simulink model "demoDPThrusterModels"  (R2022a)
settings: Solver=ode45  StartTime=0.0  StopTime=200  RelTol=1e-3  EnableMultiTasking=on
undefined symbols (not defined in the file): slcm
libraries: mssSimulink x2, simulink_extras x2
settings Model: Creator=thor  LastModifiedBy=thor
settings SolverCC: AlgebraicLoopSolver=TrustRegion
settings DataIOCC: LimitDataPoints=on  SaveFormat=Array  SignalLoggingSaveFormat=ModelDataLogs  ReturnWorkspaceOutputs=off  SignalLoggingName=sigsOut
settings OptimizationCC: InitFltsAndDblsToZero=on  LifeSpan=inf
settings DebuggingCC: SaveWithParameterizedLinksMsg=none  UnderspecifiedInitializationDetection=Classic  MergeDetectMultiDrivingBlocksExec=none  SignalResolutionControl=TryResolveAllWithWarning  MultiTaskDSMMsg=warning  MultiTaskCondExecSysMsg=none  FcnCallInpInsideContextMsg=warning  UnconnectedInputMsg=warning  UnconnectedOutputMsg=warning  UnconnectedLineMsg=warning  SFUnexpectedBacktrackingDiag=warning  SFNoUnconditionalDefaultTransitionDiag=warning  SFExecutionAtInitializationDiag=none  SFMachineParentedDataDiag=warning  ArithmeticOperatorsInVariantConditions=warning
settings HardwareCC: ProdBitPerPointer=32  ProdBitPerSizeT=32  ProdBitPerPtrDiffT=32  ProdLargestAtomicFloat=None  ProdIntDivRoundTo=Undefined  ProdEndianess=Unspecified  ProdWordSize=32  ProdHWDeviceType=32-bit Generic  TargetUnknown=on
settings ModelReferenceCC: PropagateSignalLabelsOutOfModel=off
settings RTWCC: DLArmComputeVersion=19.05
settings CodeAppCC: StateflowObjectComments=on
settings GRTTargetCC: TargetFcnLib=ansi_tfl_tmw.mat  TargetLangStandard=C89/C90 (ANSI)  ModelReferenceCompliant=off  CombineOutputUpdateFcns=off  MatFileLogging=off  GRTInterface=on
settings ConfigComp: CovMetricSettings=dw  CovSaveCumulativeToWorkspaceVar=on  CovSaveSingleToWorkspaceVar=on

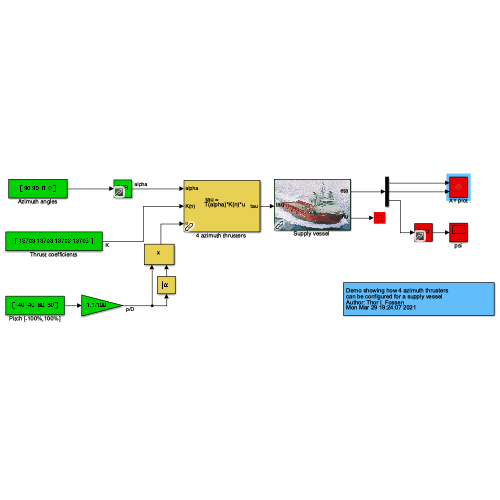
[thumbnail: Simulink's stored preview of the top-level diagram]
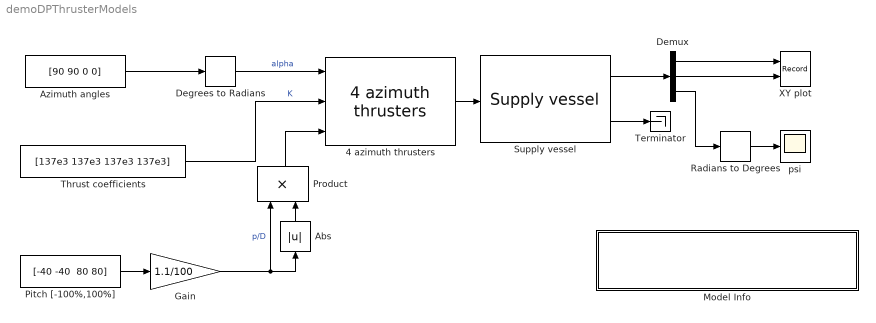
== system demoDPThrusterModels ==
  "4 azimuth thrusters " : mssSimulink/Modelling/Propulsion/Actuator Configuration/4 azimuth thrusters  SystemSampleTime=-1  VariantActivationTime=update diagram  Latency=0  AutoFrameSizeCalculation=off
  Abs : Abs
  Azimuth angles : Constant  Value=[90 90 0 0]
  Degrees to Radians : simulink_extras/Transformations/Degrees to Radians
  Demux : Demux  Outputs=3
      settings: DisplayOption=none
  Gain : Gain  Gain=1.1/100  SaturateOnIntegerOverflow=on  OutDataTypeStr=Inherit: Same as input  ParamDataTypeStr=Inherit: Same as input
  Model Info : Subsystem  LoadFcn=slcm LoadBlock;  InitFcn=slcm('UpdateAllCMBlocksInThisModelInit')  mask(CMBlock){InitialSaveTempField=, InitialBlockCM=None, BlockCM=None, Frame=on, SaveTempField=, DisplayStringWithTags=|, MaskDisplayString=Demo showing how 4 azimuth thrusters\ncan be configured for a supply vessel\nAuthor: Thor I. Fossen\nTue May 17 21:46:46 2022, HorizontalTextAlignment=Left, LeftAlignmentValue=0.02, SourceBlockDiagram=demothr, TagMaxNumber=20, CMTag1=, CMTag2=, CMTag3=, CMTag4=, CMTag5=, CMTag6=, CMTag7=, CMTag8=, CMTag9=, CMTag10=, CMTag11=, CMTag12=, CMTag13=, CMTag14=, CMTag15=, CMTag16=, CMTag17=, CMTag18=, CMTag19=, CMTag20=}
      mask DisplayStringWithTags=|
      | Demo showing how 4 azimuth thrusters
      | can be configured for a supply vessel
      | Author: Thor I. Fossen
      | %<LastModificationDate>
      mask help: This block allows revision control information to be displayed within the model.
      settings: CopyFcn=slcm CopyBlock;  DeleteFcn=slcm Cancel;  PostSaveFcn=slcm('UpdateAllCMBlocksInThisModel')  NameChangeFcn=slcm Rename;  OpenFcn=slcm
      mask Display: text(str2num(LeftAlignmentValue), 0.5, MaskDisplayString, 'HorizontalAlignment', HorizontalTextAlignment)
  Pitch [-100%,100%] : Constant  Value="[-40 -40  80 80]"
  Product : Product  SaturateOnIntegerOverflow=on  OutDataTypeStr=Inherit: Same as first input
  Radians to Degrees : simulink_extras/Transformations/Radians to Degrees
  "Supply vessel " : mssSimulink/Marine craft models/Supply vessel  D=[5.0242e4 0 0; 0 2.7229e5 -4.3933e6; 0 -4.3933e6 4.1894e8]  Minv=inv( [5.3122e6 0 0; 0 8.2831e6 0; 0 0 3.7454e9] )
  Terminator : Terminator
  Thrust coefficients : Constant  Value=[137e3 137e3 137e3 137e3]
  XY plot : Record  FileSettingsInternal="{\"entries\":[{\"content\":{\"excelSettings\":{\"content\":{},\"type\":\"Streamout.ExcelSettings\"}},\"type\":\"Streamout.FileSettingStorage\",\"uuid\":\"85dce5c7-4b4a-46ed-89de-f14b6efd32c5\"}],\"packageUris\":[\"http://schema.mathworks.com/mf0/streamout_blocks/R2020a\"],\"version\":\"1.0\"}"  Layout=[1 1]  SignalsInternal="{\"entries\":[{\"content\":{\"signals\":[{\"content\":{\"blockPath\":[\"demoDPThrusterModels/XY plot\"],\"channel\":[],\"dimensions\":[1],\"domain\":\"demoDPThrusterModels/XY plot\",\"lineColor\":\"#a2142f\",\"plots\":[1],\"port\":1,\"sid\":[\"\"],\"signalID\":721,\"signalName\":\"Demux:1\"},\"type\":\"RecordBlkView.Signal\",\"uuid\":\"12c5ca3e-2f2c-42b5-af1e-aec715ebc375\"},{\"content\":{\"blockPath\":[\"demoDPThrusterModels/XY plot\"],\"channel\":[],\"dimensions\":[1],\"domain\":\"demoDPThrusterModels/XY plot\",\"lineColor\":\"#139fff\",\"plots\":[1],\"port\":2,\"sid\":[\"\"],\"signalID\":725,\"signalName\":\"Demux:2\"},\"type\":\"RecordBlkView.Signal\",\"uuid\":\"9ca6c230-81b0-4393-8652-105309faf4e7\"}]},\"type\":\"RecordBlkView.InputSignals\",\"uuid\":\"bf2ebf43-b8ee-4bc0-9a37-ca837c9d3c7c\"}],\"packageUris\":[\"http://schema.mathworks.com/mf0/streamout_blocks/R2020a\"],\"version\":\"1.0\"}"  VisualizationBindings="{\"xyplotplugin\":{\"info\":[{\"series\":[{\"bindingParametersList\":[{\"parameter\":\"X-Axis\",\"signalID\":721,\"signalName\":\"Demux:1\"},{\"parameter\":\"Y-Axis\",\"signalID\":725,\"signalName\":\"Demux:2\"}],\"seriesID\":46517}],\"subplotID\":1}]}}"  CompatibilityTag=XY  st=-1
  psi : Scope
  wires:
  "4 azimuth thrusters "/1 -> "Supply vessel "/1
  "Supply vessel "/1 -> Demux/1
  Demux/1 -> XY plot/1
  Demux/2 -> XY plot/2
  "Supply vessel "/2 -> Terminator/1
  Degrees to Radians/1 -> "4 azimuth thrusters "/1  "alpha"
  Thrust coefficients/1 -> "4 azimuth thrusters "/2  "K"
  Pitch [-100%,100%]/1 -> Gain/1
  Abs/1 -> Product/2
  Gain/1 -> Product/1, Abs/1  "p/D"
  Product/1 -> "4 azimuth thrusters "/3
  Demux/3 -> Radians to Degrees/1
  Radians to Degrees/1 -> psi/1
  Azimuth angles/1 -> Degrees to Radians/1

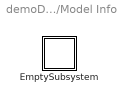
== system demoDPThrusterModels/Model Info ==
  EmptySubsystem : Subsystem

== system demoDPThrusterModels/Model Info/EmptySubsystem ==
